simulink model "D2D_PHY_SI_Simulink"  (R2024b)
settings: Solver=VariableStepAuto  StartTime=0.0  StopTime=10.0  RelTol=1e-3
model workspace (MAT data in the model file):
  d2dCfg.link.modulation = 'PAM4'
  d2dCfg.link.baud_Gbps = 56.25
  d2dCfg.link.sps = 16
  d2dCfg.link.nBits = 10000
  d2dCfg.link.skipUI = 32
  d2dCfg.link.snr_dB = 28
  d2dCfg.link.rjUI_rms = 0.005
  d2dCfg.link.djUI_pp = 0.02
  d2dCfg.link.djFreq = 0.001
  d2dCfg.link.cdrBw = 0.1
  d2dCfg.link.seed = 202409
  d2dCfg.link.lineRate_Gbps = 112.5
  d2dCfg.link.baud_GBd = 56.25
  d2dCfg.rawPcs.pattern = 'PRBS31'
  d2dCfg.rawPcs.errInject = 0
  d2dCfg.txPma.lane.txEqMain = 0.98
  d2dCfg.txPma.lane.txEqPre = 0.01
  d2dCfg.txPma.lane.txEqPost = 0.01
  d2dCfg.txPma.lane.ffeNormalize = 1
  d2dCfg.txPma.lane.amplitude = 1
  d2dCfg.txPma.lane.ffeMode = 'three_tap'
  d2dCfg.txPma.lane.ffeOffsets = [-1 0 1]
  d2dCfg.txPma.lane.ffeCoeffs = [-0.01 0.98 -0.01]
  d2dCfg.txPma.lane.ffeCurrentConstraint = 1
  d2dCfg.txPma.lane.ffe.mode = 'three_tap'
  d2dCfg.txPma.lane.ffe.offsets = [-1 0 1]
  d2dCfg.txPma.lane.ffe.coeffs = [-0.01 0.98 -0.01]
  d2dCfg.txPma.lane.ffe.normalize = 1
  d2dCfg.txPma.lane.ffe.currentConstraint = 1
  d2dCfg.txPma.lane.sixTapPreset.offsets = [-2 -1 0 1 2 3]
  d2dCfg.txPma.lane.sixTapPreset.coeffs = [-0.03 -0.05 0.88 -0.06 -0.04 -0.02]
  d2dCfg.txPma.lane.sixTapPreset.description = 'model-selected regression assumption; not paper-disclosed coefficients'
  d2dCfg.txPma.lane.enableDacQuantization = 1
  d2dCfg.txPma.lane.dacLevels = 206
  d2dCfg.txPma.lane.targetSwing = 1
  d2dCfg.txPma.lane.gainError = 0
  d2dCfg.txPma.lane.enableSwingCalibration = 1
  d2dCfg.rxPma.lane.ctleBoost_dB = 4
  d2dCfg.rxPma.lane.ctleFz = 0.25
  d2dCfg.rxPma.lane.termGain = 1
  d2dCfg.rxPma.lane.clockMode = 'forwarded'
  d2dCfg.rxPma.lane.terminationMode = 'AC'
  d2dCfg.rxPma.lane.enableAcPre = 1
  d2dCfg.rxPma.lane.enableAcPost = 1
  d2dCfg.rxPma.lane.acPreCorner_UI = 0.0003
  d2dCfg.rxPma.lane.acPostCorner_UI = 0.0003
  d2dCfg.rxPma.lane.acInitialState = 'steady_state'
  d2dCfg.rxPma.lane.enableAgc = 0
  d2dCfg.rxPma.lane.ctlePolicy = 'paper_grid'
  d2dCfg.rxPma.lane.ctleGrid_dB = [0 0.2 0.4 0.6 0.8 1 1.2 1.4 1.6 1.8 2 2.2 2.4 2.6 2.8 3 3.2 3.4 3.6 3.8 4 4.2 4.4 4.6 4.8 5 5.2 5.4 5.6 5.8 6]
  d2dCfg.rxPma.lane.ctleAppliedBoost_dB = 4
  d2dCfg.rxPma.lane.samplerRoles.enabled = 1
  d2dCfg.rxPma.lane.samplerRoles.quarterRateBranches = 4
  d2dCfg.rxPma.lane.samplerRoles.roleCounts.data = 12
  d2dCfg.rxPma.lane.samplerRoles.roleCounts.edge = 4
  d2dCfg.rxPma.lane.samplerRoles.roleCounts.spare = 4
  d2dCfg.rxPma.lane.samplerRoles.roleCounts.total = 20
  d2dCfg.rxPma.lane.samplerRoles.levelShiftCodes.data = [2 0 -2]
  d2dCfg.rxPma.lane.samplerRoles.levelShiftCodes.edge = 0
  d2dCfg.rxPma.lane.samplerRoles.levelShiftCodes.spare = [3 1 -1 -3]
  d2dCfg.rxPma.lane.samplerRoles.samplerOffsetCodes = 0
  d2dCfg.rxPma.lane.samplerRoles.thresholdAssumptions = [-2 0 2]
  d2dCfg.rxPma.lane.samplerRoles.offsetCalibrationPlaceholder = 'not implemented in Stage D'
  d2dCfg.rxPma.lane.acSelectedCorner_UI = 0.0003
  d2dCfg.rxPma.lane.acSelectionBasis = 'bounded cycles/UI sweep; maximize valid received eye margin; no BER optimization'
  d2dCfg.channel.lossNyq_dB = 8
  d2dCfg.channel.poles = 3
  d2dCfg.channel.mode = 'analytic_il'
  d2dCfg.channel.refFreq_GHz = 28
  d2dCfg.channel.baud_GBd = 56.25
  d2dCfg.channel.lossAtRef_dB = 8
  d2dCfg.channel.lossSweep_dB = [0.5 2 4 6 8 10]
  d2dCfg.paper.id = 'VLSI2024_XSR_3nm'
  d2dCfg.paper.preset = 'VLSI Typical'
  d2dCfg.paper.mode = 'link_behavioral'
  d2dCfg.paper.rateRange_Gbps = [9.8 113]
  d2dCfg.paper.txEyeRate_Gbps = 112.5
  d2dCfg.paper.berRate_Gbps = 112
  d2dCfg.paper.headlineRate_Gbps = 113
  d2dCfg.paper.rateContext.range_Gbps = [9.8 113]
  d2dCfg.paper.rateContext.txEye_Gbps = 112.5
  d2dCfg.paper.rateContext.ber_Gbps = 112
  d2dCfg.paper.rateContext.headlineTable_Gbps = 113
  d2dCfg.paper.facts.packageTopology = '2D/2.5D CoWoS'
  d2dCfg.paper.facts.channelLength_mm = [1 80]
  d2dCfg.paper.facts.nextAt28GHz_dB = -40
  d2dCfg.paper.facts.fextAt28GHz_dB = -38
  d2dCfg.paper.facts.next_dB = -40
  d2dCfg.paper.facts.fext_dB = -38
  d2dCfg.paper.facts.quotedEnergy_pJ_per_bit = 0.9
  d2dCfg.paper.facts.dacLevels = 206
  d2dCfg.paper.facts.energy_pJ_per_bit = 0.9
  d2dCfg.paper.facts.ctleMaxBoost_dB = 6
  d2dCfg.paper.facts.ctleMaxStep_dB = 0.2
  d2dCfg.paper.facts.samplerRoleCounts.data = 12
  d2dCfg.paper.facts.samplerRoleCounts.edge = 4
  d2dCfg.paper.facts.samplerRoleCounts.spare = 4
  d2dCfg.paper.facts.samplerRoleCounts.total = 20
  d2dCfg.paper.facts.dllCount = 2
  d2dCfg.paper.facts.piCount = 1
  d2dCfg.paper.facts.piInlDnl = '< +/-0.5 LSB'
  d2dCfg.paper.facts.piInlDnl_LSB = '< +/-0.5 LSB'
  d2dCfg.paper.facts.pllTxIntegratedJitter_fs = 194
  d2dCfg.paper.facts.pllTxIntegratedJitter_UI = 0.0109125
  d2dCfg.paper.facts.pllTxIntegratedJitterContext = 'PLL+TX integrated; filter/measurement context'
  d2dCfg.paper.facts.table1LossAtRef_dB = 10.8
  d2dCfg.paper.facts.table1Loss_dB = 10.8
  d2dCfg.paper.facts.table1_IL_dB = 10.8
  d2dCfg.paper.assumptions.channelModel = 'calibrated analytic_il at 28 GHz; no real S-parameters'
  d2dCfg.paper.assumptions.quotedEnergyScope = 'quoted only; not a model prediction'
  d2dCfg.paper.assumptions.crosstalk = 'NEXT/FEXT facts recorded; MIMO crosstalk unmodeled'
  d2dCfg.phy.nLane = 8
  d2dCfg.model.useReferenceAlign = 0
  d2dCfg.model.useManualPhase = 0
  d2dCfg.model.manualPhaseUI = 0.5
  d2dCfg.model.manualDelayUI = 0
  d2dCfg.model.enablePaperAdaptation = 0
  d2dCfg.model.trainingMode = 'decision_directed'
  d2dCfg.model.cdrOptions.nCodes = 64
  d2dCfg.model.cdrOptions.initialPhaseUI = 0.5
  d2dCfg.model.cdrOptions.loopGainCodes = 1
  d2dCfg.model.cdrOptions.loopBandwidthProxy = 0.015625
  d2dCfg.model.cdrOptions.updateCadence = 1
  d2dCfg.model.cdrOptions.lockWindow = 32
  d2dCfg.model.cdrOptions.lockToleranceUI = 0.08
  d2dCfg.model.cdrOptions.mismatchBoundLSB = 0.49
  d2dCfg.model.cdrOptions.mismatchSeed = 202409
  d2dCfg.model.cdrOptions.enabled = 1
  d2dCfg.model.cdrOptions.maxStepCodes = 2
  d2dCfg.model.debugStages.startupCalibration = 1
  d2dCfg.model.debugStages.ctleTraining = 1
  d2dCfg.model.debugStages.ffeTraining = 1
  d2dCfg.model.debugStages.samplerCalibration = 1
  d2dCfg.model.debugStages.clockTraining = 1
  d2dCfg.model.debugStages.cdrEnabled = 1
  d2dCfg.model.debugStages.startupCalibrationBudgetUI = 64
  d2dCfg.model.debugStages.ctleTrainingBudgetUI = 128
  d2dCfg.model.debugStages.ffeTrainingBudgetUI = 128
  d2dCfg.model.debugStages.samplerCalibrationBudgetUI = 64
  d2dCfg.model.debugStages.clockTrainingBudgetUI = 64
  d2dCfg.model.debugStages.postLockWaitUI = 16
  d2dCfg.model.debugOptions.postLockWaitUI = 16
  d2dCfg.model.debugOptions.preLockSentinel = NaN
  d2dCfg.model.resultRoot = 'results/vlsi2024_xsr'
undefined symbols (not defined in the file or in its folder): dspChannel, dspCtle, dspFfeVector, dspMap, dspPam4Leveling, dspPaperCdr, dspPaperDriver, dspSample, dspSlice, repelem
settings Model: Creator=ahu161  LastModifiedBy=ahu161

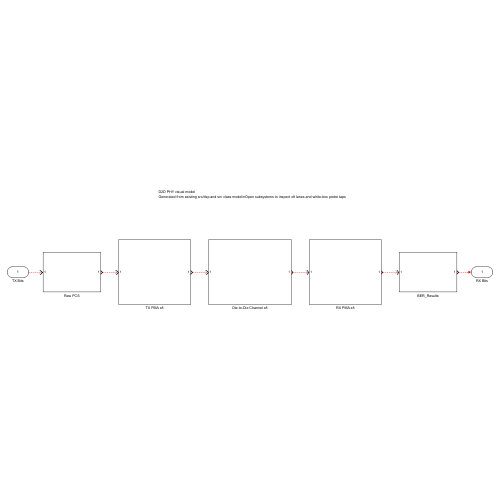
[thumbnail: Simulink's stored preview of the top-level diagram]
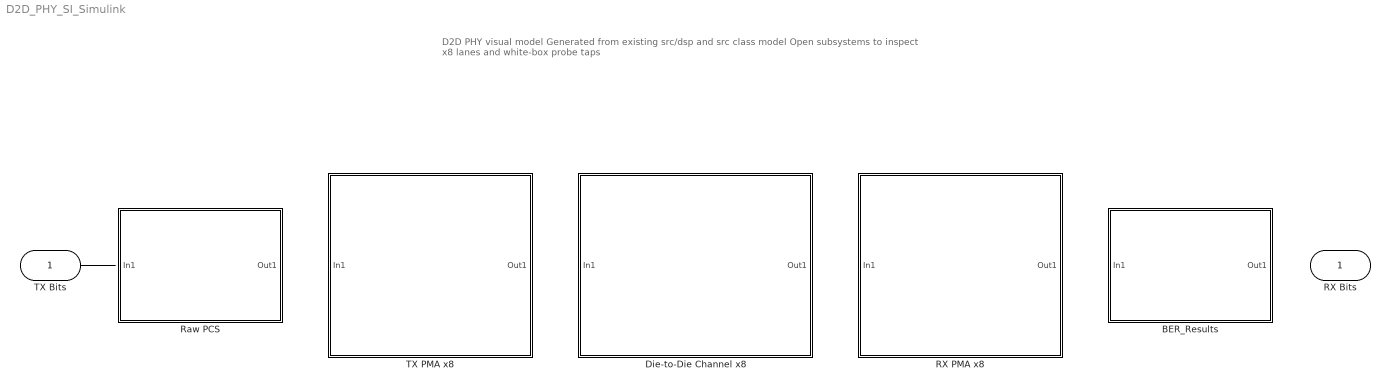
== system D2D_PHY_SI_Simulink ==
  note: D2D PHY visual model
      | Generated from existing src/dsp and src class model\nOpen subsystems to inspect x8 lanes and white-box probe taps
  TX Bits : Inport
  BER_Results : Subsystem
  Die-to-Die Channel x8 : Subsystem
  RX PMA x8 : Subsystem
  Raw PCS : Subsystem
  TX PMA x8 : Subsystem
  RX Bits : Outport
  wires:
  TX Bits/1 -> ?
  ? -> ?
  ? -> ?
  ? -> ?
  ? -> ?
  ? -> RX Bits/1

== system D2D_PHY_SI_Simulink/BER_Results ==
  In1 : Inport
  BER calculator : MATLABFcn  MATLABFcn=mean(u~=0)
  BER result : ToWorkspace  VariableName=simulinkBer  SampleTime=-1
  Out1 : Outport
  wires:
  In1/1 -> BER calculator/1
  BER calculator/1 -> BER result/1, Out1/1

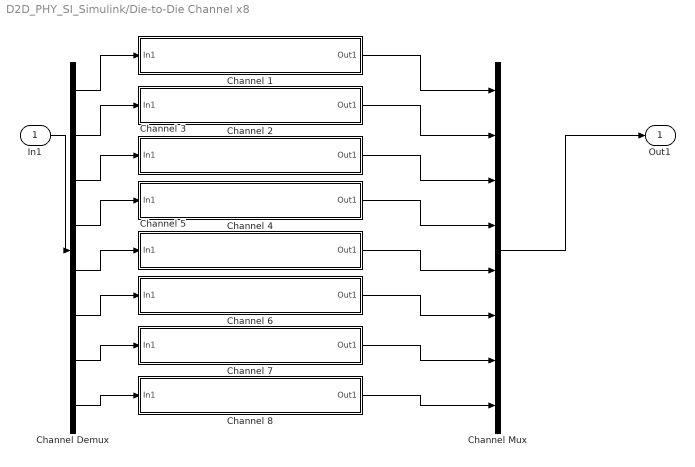
== system D2D_PHY_SI_Simulink/Die-to-Die Channel x8 ==
  In1 : Inport
  Channel 1 : Subsystem
  Channel 2 : Subsystem
  Channel 3 : Subsystem
  Channel 4 : Subsystem
  Channel 5 : Subsystem
  Channel 6 : Subsystem
  Channel 7 : Subsystem
  Channel 8 : Subsystem
  Channel Demux : Demux  Outputs=8
  Channel Mux : Mux  Inputs=8
  Out1 : Outport
  wires:
  In1/1 -> Channel Demux/1
  Channel Demux/1 -> Channel 1/1(In1)
  Channel 1/1(Out1) -> Channel Mux/1
  Channel Demux/2 -> Channel 2/1(In1)
  Channel 2/1(Out1) -> Channel Mux/2
  Channel Demux/3 -> Channel 3/1(In1)
  Channel 3/1(Out1) -> Channel Mux/3
  Channel Demux/4 -> Channel 4/1(In1)
  Channel 4/1(Out1) -> Channel Mux/4
  Channel Demux/5 -> Channel 5/1(In1)
  Channel 5/1(Out1) -> Channel Mux/5
  Channel Demux/6 -> Channel 6/1(In1)
  Channel 6/1(Out1) -> Channel Mux/6
  Channel Demux/7 -> Channel 7/1(In1)
  Channel 7/1(Out1) -> Channel Mux/7
  Channel Demux/8 -> Channel 8/1(In1)
  Channel 8/1(Out1) -> Channel Mux/8
  Channel Mux/1 -> Out1/1

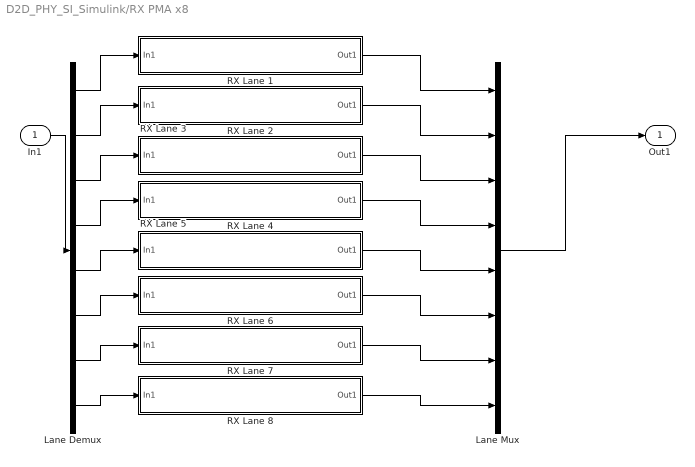
== system D2D_PHY_SI_Simulink/RX PMA x8 ==
  In1 : Inport
  Lane Demux : Demux  Outputs=8
  Lane Mux : Mux  Inputs=8
  RX Lane 1 : Subsystem
  RX Lane 2 : Subsystem
  RX Lane 3 : Subsystem
  RX Lane 4 : Subsystem
  RX Lane 5 : Subsystem
  RX Lane 6 : Subsystem
  RX Lane 7 : Subsystem
  RX Lane 8 : Subsystem
  Out1 : Outport
  wires:
  In1/1 -> Lane Demux/1
  Lane Demux/1 -> RX Lane 1/1(In1)
  RX Lane 1/1(Out1) -> Lane Mux/1
  Lane Demux/2 -> RX Lane 2/1(In1)
  RX Lane 2/1(Out1) -> Lane Mux/2
  Lane Demux/3 -> RX Lane 3/1(In1)
  RX Lane 3/1(Out1) -> Lane Mux/3
  Lane Demux/4 -> RX Lane 4/1(In1)
  RX Lane 4/1(Out1) -> Lane Mux/4
  Lane Demux/5 -> RX Lane 5/1(In1)
  RX Lane 5/1(Out1) -> Lane Mux/5
  Lane Demux/6 -> RX Lane 6/1(In1)
  RX Lane 6/1(Out1) -> Lane Mux/6
  Lane Demux/7 -> RX Lane 7/1(In1)
  RX Lane 7/1(Out1) -> Lane Mux/7
  Lane Demux/8 -> RX Lane 8/1(In1)
  RX Lane 8/1(Out1) -> Lane Mux/8
  Lane Mux/1 -> Out1/1

== system D2D_PHY_SI_Simulink/Raw PCS ==
  In1 : Inport
  dspPrbs_Pattern_Source : MATLABFcn  MATLABFcn=dspMap(u,d2dCfg.link.modulation)
  Out1 : Outport
  wires:
  In1/1 -> dspPrbs_Pattern_Source/1
  dspPrbs_Pattern_Source/1 -> [rawPcs_rxBits], Out1/1

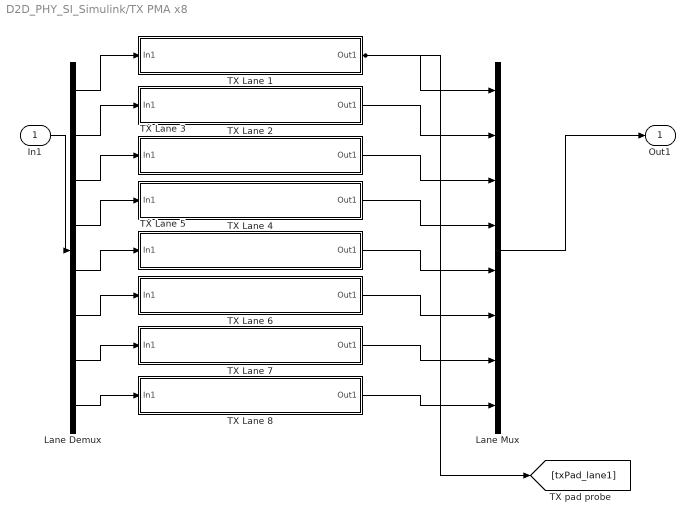
== system D2D_PHY_SI_Simulink/TX PMA x8 ==
  In1 : Inport
  Lane Demux : Demux  Outputs=8
  Lane Mux : Mux  Inputs=8
  TX Lane 1 : Subsystem
  TX Lane 2 : Subsystem
  TX Lane 3 : Subsystem
  TX Lane 4 : Subsystem
  TX Lane 5 : Subsystem
  TX Lane 6 : Subsystem
  TX Lane 7 : Subsystem
  TX Lane 8 : Subsystem
  Out1 : Outport
  wires:
  In1/1 -> Lane Demux/1
  Lane Demux/1 -> TX Lane 1/1(In1)
  TX Lane 1/1(Out1) -> Lane Mux/1, [txPad_lane1]
  Lane Demux/2 -> TX Lane 2/1(In1)
  TX Lane 2/1(Out1) -> Lane Mux/2
  Lane Demux/3 -> TX Lane 3/1(In1)
  TX Lane 3/1(Out1) -> Lane Mux/3
  Lane Demux/4 -> TX Lane 4/1(In1)
  TX Lane 4/1(Out1) -> Lane Mux/4
  Lane Demux/5 -> TX Lane 5/1(In1)
  TX Lane 5/1(Out1) -> Lane Mux/5
  Lane Demux/6 -> TX Lane 6/1(In1)
  TX Lane 6/1(Out1) -> Lane Mux/6
  Lane Demux/7 -> TX Lane 7/1(In1)
  TX Lane 7/1(Out1) -> Lane Mux/7
  Lane Demux/8 -> TX Lane 8/1(In1)
  TX Lane 8/1(Out1) -> Lane Mux/8
  Lane Mux/1 -> Out1/1

== system D2D_PHY_SI_Simulink/Die-to-Die Channel x8/Channel 1 ==
  In1 : Inport
  dspChannel : MATLABFcn  MATLABFcn=dspChannel(u,d2dCfg.link.sps,d2dCfg.channel.lossAtRef_dB,d2dCfg.channel.poles,struct('mode',d2dCfg.channel.mode,'refFreq_GHz',d2dCfg.channel.refFreq_GHz,'baud_GBd',d2dCfg.channel.baud_GBd,'lossAtRef_dB',d2dCfg.channel.lossAtRef_dB))
  Out1 : Outport
  wires:
  In1/1 -> dspChannel/1
  dspChannel/1 -> Out1/1

== system D2D_PHY_SI_Simulink/Die-to-Die Channel x8/Channel 2 ==
  In1 : Inport
  dspChannel : MATLABFcn  MATLABFcn=dspChannel(u,d2dCfg.link.sps,d2dCfg.channel.lossAtRef_dB,d2dCfg.channel.poles,struct('mode',d2dCfg.channel.mode,'refFreq_GHz',d2dCfg.channel.refFreq_GHz,'baud_GBd',d2dCfg.channel.baud_GBd,'lossAtRef_dB',d2dCfg.channel.lossAtRef_dB))
  Out1 : Outport
  wires:
  In1/1 -> dspChannel/1
  dspChannel/1 -> Out1/1

== system D2D_PHY_SI_Simulink/Die-to-Die Channel x8/Channel 3 ==
  In1 : Inport
  dspChannel : MATLABFcn  MATLABFcn=dspChannel(u,d2dCfg.link.sps,d2dCfg.channel.lossAtRef_dB,d2dCfg.channel.poles,struct('mode',d2dCfg.channel.mode,'refFreq_GHz',d2dCfg.channel.refFreq_GHz,'baud_GBd',d2dCfg.channel.baud_GBd,'lossAtRef_dB',d2dCfg.channel.lossAtRef_dB))
  Out1 : Outport
  wires:
  In1/1 -> dspChannel/1
  dspChannel/1 -> Out1/1

== system D2D_PHY_SI_Simulink/Die-to-Die Channel x8/Channel 4 ==
  In1 : Inport
  dspChannel : MATLABFcn  MATLABFcn=dspChannel(u,d2dCfg.link.sps,d2dCfg.channel.lossAtRef_dB,d2dCfg.channel.poles,struct('mode',d2dCfg.channel.mode,'refFreq_GHz',d2dCfg.channel.refFreq_GHz,'baud_GBd',d2dCfg.channel.baud_GBd,'lossAtRef_dB',d2dCfg.channel.lossAtRef_dB))
  Out1 : Outport
  wires:
  In1/1 -> dspChannel/1
  dspChannel/1 -> Out1/1

== system D2D_PHY_SI_Simulink/Die-to-Die Channel x8/Channel 5 ==
  In1 : Inport
  dspChannel : MATLABFcn  MATLABFcn=dspChannel(u,d2dCfg.link.sps,d2dCfg.channel.lossAtRef_dB,d2dCfg.channel.poles,struct('mode',d2dCfg.channel.mode,'refFreq_GHz',d2dCfg.channel.refFreq_GHz,'baud_GBd',d2dCfg.channel.baud_GBd,'lossAtRef_dB',d2dCfg.channel.lossAtRef_dB))
  Out1 : Outport
  wires:
  In1/1 -> dspChannel/1
  dspChannel/1 -> Out1/1

== system D2D_PHY_SI_Simulink/Die-to-Die Channel x8/Channel 6 ==
  In1 : Inport
  dspChannel : MATLABFcn  MATLABFcn=dspChannel(u,d2dCfg.link.sps,d2dCfg.channel.lossAtRef_dB,d2dCfg.channel.poles,struct('mode',d2dCfg.channel.mode,'refFreq_GHz',d2dCfg.channel.refFreq_GHz,'baud_GBd',d2dCfg.channel.baud_GBd,'lossAtRef_dB',d2dCfg.channel.lossAtRef_dB))
  Out1 : Outport
  wires:
  In1/1 -> dspChannel/1
  dspChannel/1 -> Out1/1

== system D2D_PHY_SI_Simulink/Die-to-Die Channel x8/Channel 7 ==
  In1 : Inport
  dspChannel : MATLABFcn  MATLABFcn=dspChannel(u,d2dCfg.link.sps,d2dCfg.channel.lossAtRef_dB,d2dCfg.channel.poles,struct('mode',d2dCfg.channel.mode,'refFreq_GHz',d2dCfg.channel.refFreq_GHz,'baud_GBd',d2dCfg.channel.baud_GBd,'lossAtRef_dB',d2dCfg.channel.lossAtRef_dB))
  Out1 : Outport
  wires:
  In1/1 -> dspChannel/1
  dspChannel/1 -> Out1/1

== system D2D_PHY_SI_Simulink/Die-to-Die Channel x8/Channel 8 ==
  In1 : Inport
  dspChannel : MATLABFcn  MATLABFcn=dspChannel(u,d2dCfg.link.sps,d2dCfg.channel.lossAtRef_dB,d2dCfg.channel.poles,struct('mode',d2dCfg.channel.mode,'refFreq_GHz',d2dCfg.channel.refFreq_GHz,'baud_GBd',d2dCfg.channel.baud_GBd,'lossAtRef_dB',d2dCfg.channel.lossAtRef_dB))
  Out1 : Outport
  wires:
  In1/1 -> dspChannel/1
  dspChannel/1 -> Out1/1

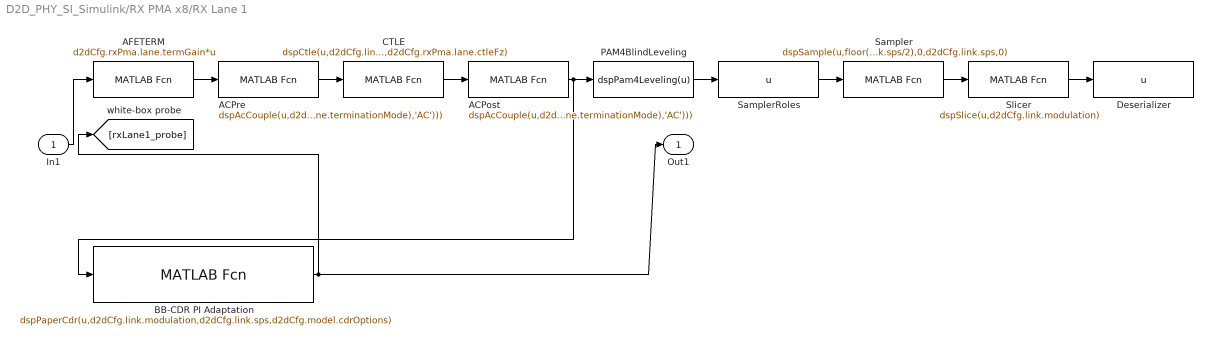
== system D2D_PHY_SI_Simulink/RX PMA x8/RX Lane 1 ==
  In1 : Inport
  ACPost : MATLABFcn  MATLABFcn=dspAcCouple(u,d2dCfg.link.sps,d2dCfg.rxPma.lane.acPostCorner_UI,struct('enabled',d2dCfg.rxPma.lane.enableAcPost && strcmpi(char(d2dCfg.rxPma.lane.terminationMode),'AC')))
  ACPre : MATLABFcn  MATLABFcn=dspAcCouple(u,d2dCfg.link.sps,d2dCfg.rxPma.lane.acPreCorner_UI,struct('enabled',d2dCfg.rxPma.lane.enableAcPre && strcmpi(char(d2dCfg.rxPma.lane.terminationMode),'AC')))
  AFETERM : MATLABFcn  MATLABFcn=d2dCfg.rxPma.lane.termGain*u
  BB-CDR PI Adaptation : MATLABFcn  MATLABFcn=dspPaperCdr(u,d2dCfg.link.modulation,d2dCfg.link.sps,d2dCfg.model.cdrOptions)
  CTLE : MATLABFcn  MATLABFcn=dspCtle(u,d2dCfg.link.sps,d2dCfg.rxPma.lane.ctleBoost_dB,d2dCfg.rxPma.lane.ctleFz)
  Deserializer : MATLABFcn  MATLABFcn=u
  PAM4BlindLeveling : MATLABFcn  MATLABFcn=dspPam4Leveling(u)
  Sampler : MATLABFcn  MATLABFcn=dspSample(u,floor(d2dCfg.link.sps/2),0,d2dCfg.link.sps,0)
  SamplerRoles : MATLABFcn  MATLABFcn=u
  Slicer : MATLABFcn  MATLABFcn=dspSlice(u,d2dCfg.link.modulation)
  Out1 : Outport
  wires:
  In1/1 -> AFETERM/1
  AFETERM/1 -> ACPre/1
  ACPre/1 -> CTLE/1
  CTLE/1 -> ACPost/1
  ACPost/1 -> PAM4BlindLeveling/1, BB-CDR PI Adaptation/1
  PAM4BlindLeveling/1 -> SamplerRoles/1
  SamplerRoles/1 -> Sampler/1
  Sampler/1 -> Slicer/1
  Slicer/1 -> Deserializer/1
  BB-CDR PI Adaptation/1 -> Out1/1, [rxLane1_probe]

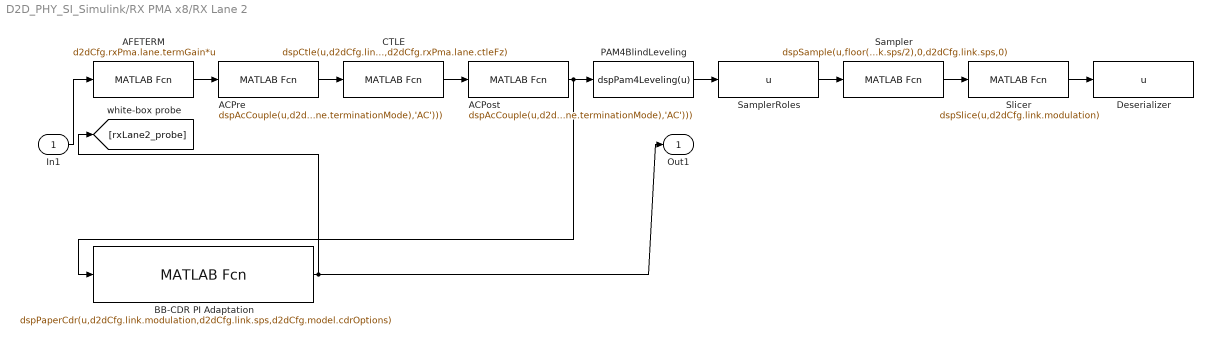
== system D2D_PHY_SI_Simulink/RX PMA x8/RX Lane 2 ==
  In1 : Inport
  ACPost : MATLABFcn  MATLABFcn=dspAcCouple(u,d2dCfg.link.sps,d2dCfg.rxPma.lane.acPostCorner_UI,struct('enabled',d2dCfg.rxPma.lane.enableAcPost && strcmpi(char(d2dCfg.rxPma.lane.terminationMode),'AC')))
  ACPre : MATLABFcn  MATLABFcn=dspAcCouple(u,d2dCfg.link.sps,d2dCfg.rxPma.lane.acPreCorner_UI,struct('enabled',d2dCfg.rxPma.lane.enableAcPre && strcmpi(char(d2dCfg.rxPma.lane.terminationMode),'AC')))
  AFETERM : MATLABFcn  MATLABFcn=d2dCfg.rxPma.lane.termGain*u
  BB-CDR PI Adaptation : MATLABFcn  MATLABFcn=dspPaperCdr(u,d2dCfg.link.modulation,d2dCfg.link.sps,d2dCfg.model.cdrOptions)
  CTLE : MATLABFcn  MATLABFcn=dspCtle(u,d2dCfg.link.sps,d2dCfg.rxPma.lane.ctleBoost_dB,d2dCfg.rxPma.lane.ctleFz)
  Deserializer : MATLABFcn  MATLABFcn=u
  PAM4BlindLeveling : MATLABFcn  MATLABFcn=dspPam4Leveling(u)
  Sampler : MATLABFcn  MATLABFcn=dspSample(u,floor(d2dCfg.link.sps/2),0,d2dCfg.link.sps,0)
  SamplerRoles : MATLABFcn  MATLABFcn=u
  Slicer : MATLABFcn  MATLABFcn=dspSlice(u,d2dCfg.link.modulation)
  Out1 : Outport
  wires:
  In1/1 -> AFETERM/1
  AFETERM/1 -> ACPre/1
  ACPre/1 -> CTLE/1
  CTLE/1 -> ACPost/1
  ACPost/1 -> PAM4BlindLeveling/1, BB-CDR PI Adaptation/1
  PAM4BlindLeveling/1 -> SamplerRoles/1
  SamplerRoles/1 -> Sampler/1
  Sampler/1 -> Slicer/1
  Slicer/1 -> Deserializer/1
  BB-CDR PI Adaptation/1 -> Out1/1, [rxLane2_probe]

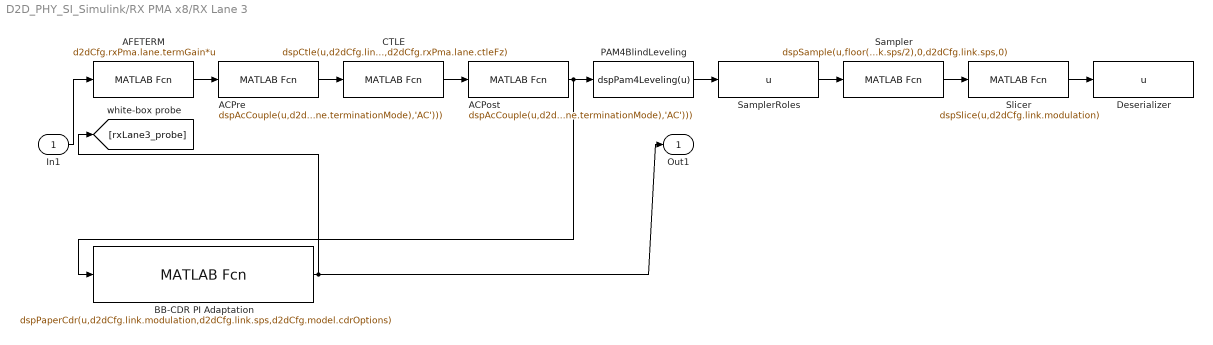
== system D2D_PHY_SI_Simulink/RX PMA x8/RX Lane 3 ==
  In1 : Inport
  ACPost : MATLABFcn  MATLABFcn=dspAcCouple(u,d2dCfg.link.sps,d2dCfg.rxPma.lane.acPostCorner_UI,struct('enabled',d2dCfg.rxPma.lane.enableAcPost && strcmpi(char(d2dCfg.rxPma.lane.terminationMode),'AC')))
  ACPre : MATLABFcn  MATLABFcn=dspAcCouple(u,d2dCfg.link.sps,d2dCfg.rxPma.lane.acPreCorner_UI,struct('enabled',d2dCfg.rxPma.lane.enableAcPre && strcmpi(char(d2dCfg.rxPma.lane.terminationMode),'AC')))
  AFETERM : MATLABFcn  MATLABFcn=d2dCfg.rxPma.lane.termGain*u
  BB-CDR PI Adaptation : MATLABFcn  MATLABFcn=dspPaperCdr(u,d2dCfg.link.modulation,d2dCfg.link.sps,d2dCfg.model.cdrOptions)
  CTLE : MATLABFcn  MATLABFcn=dspCtle(u,d2dCfg.link.sps,d2dCfg.rxPma.lane.ctleBoost_dB,d2dCfg.rxPma.lane.ctleFz)
  Deserializer : MATLABFcn  MATLABFcn=u
  PAM4BlindLeveling : MATLABFcn  MATLABFcn=dspPam4Leveling(u)
  Sampler : MATLABFcn  MATLABFcn=dspSample(u,floor(d2dCfg.link.sps/2),0,d2dCfg.link.sps,0)
  SamplerRoles : MATLABFcn  MATLABFcn=u
  Slicer : MATLABFcn  MATLABFcn=dspSlice(u,d2dCfg.link.modulation)
  Out1 : Outport
  wires:
  In1/1 -> AFETERM/1
  AFETERM/1 -> ACPre/1
  ACPre/1 -> CTLE/1
  CTLE/1 -> ACPost/1
  ACPost/1 -> PAM4BlindLeveling/1, BB-CDR PI Adaptation/1
  PAM4BlindLeveling/1 -> SamplerRoles/1
  SamplerRoles/1 -> Sampler/1
  Sampler/1 -> Slicer/1
  Slicer/1 -> Deserializer/1
  BB-CDR PI Adaptation/1 -> Out1/1, [rxLane3_probe]

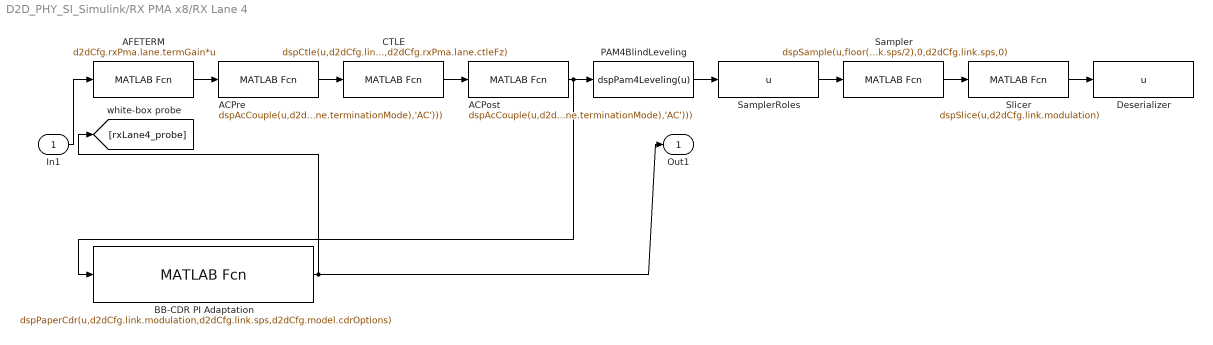
== system D2D_PHY_SI_Simulink/RX PMA x8/RX Lane 4 ==
  In1 : Inport
  ACPost : MATLABFcn  MATLABFcn=dspAcCouple(u,d2dCfg.link.sps,d2dCfg.rxPma.lane.acPostCorner_UI,struct('enabled',d2dCfg.rxPma.lane.enableAcPost && strcmpi(char(d2dCfg.rxPma.lane.terminationMode),'AC')))
  ACPre : MATLABFcn  MATLABFcn=dspAcCouple(u,d2dCfg.link.sps,d2dCfg.rxPma.lane.acPreCorner_UI,struct('enabled',d2dCfg.rxPma.lane.enableAcPre && strcmpi(char(d2dCfg.rxPma.lane.terminationMode),'AC')))
  AFETERM : MATLABFcn  MATLABFcn=d2dCfg.rxPma.lane.termGain*u
  BB-CDR PI Adaptation : MATLABFcn  MATLABFcn=dspPaperCdr(u,d2dCfg.link.modulation,d2dCfg.link.sps,d2dCfg.model.cdrOptions)
  CTLE : MATLABFcn  MATLABFcn=dspCtle(u,d2dCfg.link.sps,d2dCfg.rxPma.lane.ctleBoost_dB,d2dCfg.rxPma.lane.ctleFz)
  Deserializer : MATLABFcn  MATLABFcn=u
  PAM4BlindLeveling : MATLABFcn  MATLABFcn=dspPam4Leveling(u)
  Sampler : MATLABFcn  MATLABFcn=dspSample(u,floor(d2dCfg.link.sps/2),0,d2dCfg.link.sps,0)
  SamplerRoles : MATLABFcn  MATLABFcn=u
  Slicer : MATLABFcn  MATLABFcn=dspSlice(u,d2dCfg.link.modulation)
  Out1 : Outport
  wires:
  In1/1 -> AFETERM/1
  AFETERM/1 -> ACPre/1
  ACPre/1 -> CTLE/1
  CTLE/1 -> ACPost/1
  ACPost/1 -> PAM4BlindLeveling/1, BB-CDR PI Adaptation/1
  PAM4BlindLeveling/1 -> SamplerRoles/1
  SamplerRoles/1 -> Sampler/1
  Sampler/1 -> Slicer/1
  Slicer/1 -> Deserializer/1
  BB-CDR PI Adaptation/1 -> Out1/1, [rxLane4_probe]

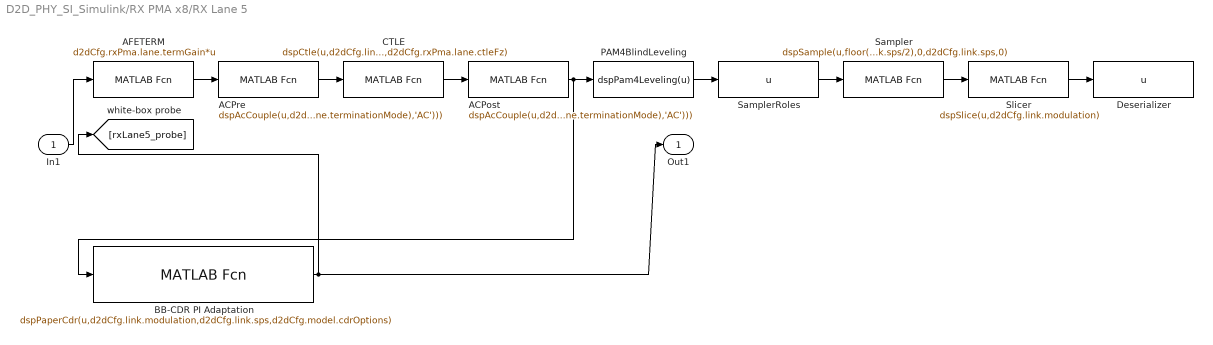
== system D2D_PHY_SI_Simulink/RX PMA x8/RX Lane 5 ==
  In1 : Inport
  ACPost : MATLABFcn  MATLABFcn=dspAcCouple(u,d2dCfg.link.sps,d2dCfg.rxPma.lane.acPostCorner_UI,struct('enabled',d2dCfg.rxPma.lane.enableAcPost && strcmpi(char(d2dCfg.rxPma.lane.terminationMode),'AC')))
  ACPre : MATLABFcn  MATLABFcn=dspAcCouple(u,d2dCfg.link.sps,d2dCfg.rxPma.lane.acPreCorner_UI,struct('enabled',d2dCfg.rxPma.lane.enableAcPre && strcmpi(char(d2dCfg.rxPma.lane.terminationMode),'AC')))
  AFETERM : MATLABFcn  MATLABFcn=d2dCfg.rxPma.lane.termGain*u
  BB-CDR PI Adaptation : MATLABFcn  MATLABFcn=dspPaperCdr(u,d2dCfg.link.modulation,d2dCfg.link.sps,d2dCfg.model.cdrOptions)
  CTLE : MATLABFcn  MATLABFcn=dspCtle(u,d2dCfg.link.sps,d2dCfg.rxPma.lane.ctleBoost_dB,d2dCfg.rxPma.lane.ctleFz)
  Deserializer : MATLABFcn  MATLABFcn=u
  PAM4BlindLeveling : MATLABFcn  MATLABFcn=dspPam4Leveling(u)
  Sampler : MATLABFcn  MATLABFcn=dspSample(u,floor(d2dCfg.link.sps/2),0,d2dCfg.link.sps,0)
  SamplerRoles : MATLABFcn  MATLABFcn=u
  Slicer : MATLABFcn  MATLABFcn=dspSlice(u,d2dCfg.link.modulation)
  Out1 : Outport
  wires:
  In1/1 -> AFETERM/1
  AFETERM/1 -> ACPre/1
  ACPre/1 -> CTLE/1
  CTLE/1 -> ACPost/1
  ACPost/1 -> PAM4BlindLeveling/1, BB-CDR PI Adaptation/1
  PAM4BlindLeveling/1 -> SamplerRoles/1
  SamplerRoles/1 -> Sampler/1
  Sampler/1 -> Slicer/1
  Slicer/1 -> Deserializer/1
  BB-CDR PI Adaptation/1 -> Out1/1, [rxLane5_probe]

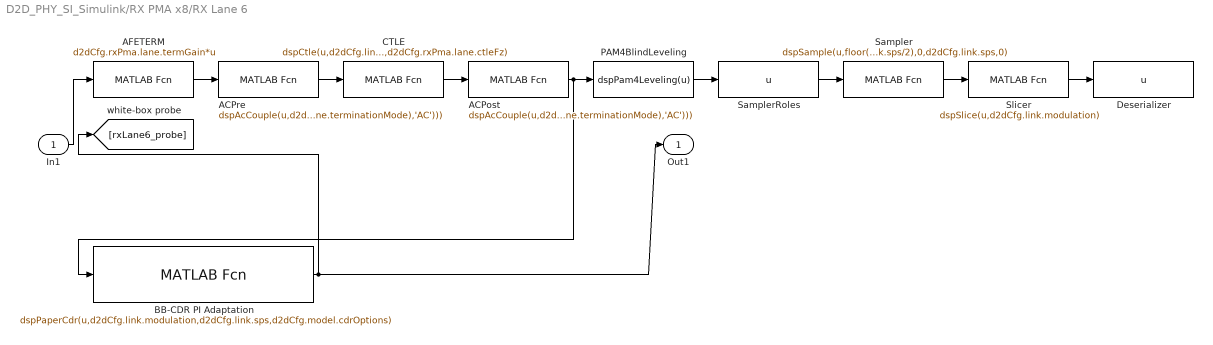
== system D2D_PHY_SI_Simulink/RX PMA x8/RX Lane 6 ==
  In1 : Inport
  ACPost : MATLABFcn  MATLABFcn=dspAcCouple(u,d2dCfg.link.sps,d2dCfg.rxPma.lane.acPostCorner_UI,struct('enabled',d2dCfg.rxPma.lane.enableAcPost && strcmpi(char(d2dCfg.rxPma.lane.terminationMode),'AC')))
  ACPre : MATLABFcn  MATLABFcn=dspAcCouple(u,d2dCfg.link.sps,d2dCfg.rxPma.lane.acPreCorner_UI,struct('enabled',d2dCfg.rxPma.lane.enableAcPre && strcmpi(char(d2dCfg.rxPma.lane.terminationMode),'AC')))
  AFETERM : MATLABFcn  MATLABFcn=d2dCfg.rxPma.lane.termGain*u
  BB-CDR PI Adaptation : MATLABFcn  MATLABFcn=dspPaperCdr(u,d2dCfg.link.modulation,d2dCfg.link.sps,d2dCfg.model.cdrOptions)
  CTLE : MATLABFcn  MATLABFcn=dspCtle(u,d2dCfg.link.sps,d2dCfg.rxPma.lane.ctleBoost_dB,d2dCfg.rxPma.lane.ctleFz)
  Deserializer : MATLABFcn  MATLABFcn=u
  PAM4BlindLeveling : MATLABFcn  MATLABFcn=dspPam4Leveling(u)
  Sampler : MATLABFcn  MATLABFcn=dspSample(u,floor(d2dCfg.link.sps/2),0,d2dCfg.link.sps,0)
  SamplerRoles : MATLABFcn  MATLABFcn=u
  Slicer : MATLABFcn  MATLABFcn=dspSlice(u,d2dCfg.link.modulation)
  Out1 : Outport
  wires:
  In1/1 -> AFETERM/1
  AFETERM/1 -> ACPre/1
  ACPre/1 -> CTLE/1
  CTLE/1 -> ACPost/1
  ACPost/1 -> PAM4BlindLeveling/1, BB-CDR PI Adaptation/1
  PAM4BlindLeveling/1 -> SamplerRoles/1
  SamplerRoles/1 -> Sampler/1
  Sampler/1 -> Slicer/1
  Slicer/1 -> Deserializer/1
  BB-CDR PI Adaptation/1 -> Out1/1, [rxLane6_probe]

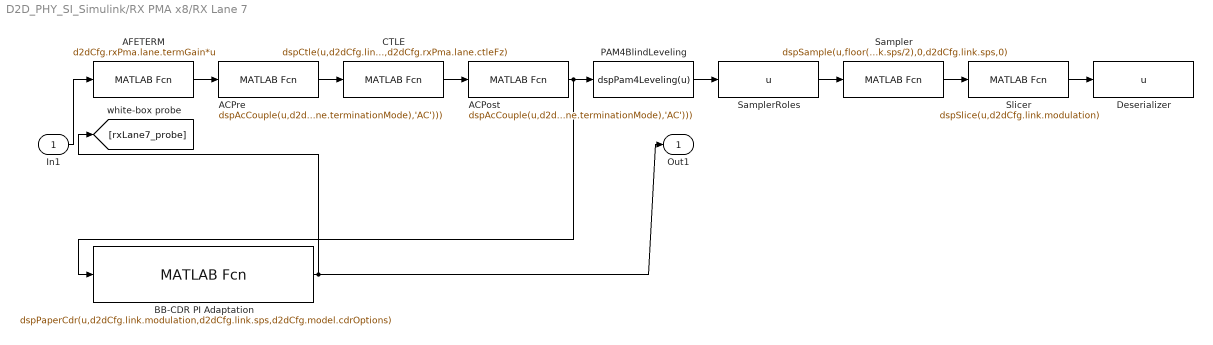
== system D2D_PHY_SI_Simulink/RX PMA x8/RX Lane 7 ==
  In1 : Inport
  ACPost : MATLABFcn  MATLABFcn=dspAcCouple(u,d2dCfg.link.sps,d2dCfg.rxPma.lane.acPostCorner_UI,struct('enabled',d2dCfg.rxPma.lane.enableAcPost && strcmpi(char(d2dCfg.rxPma.lane.terminationMode),'AC')))
  ACPre : MATLABFcn  MATLABFcn=dspAcCouple(u,d2dCfg.link.sps,d2dCfg.rxPma.lane.acPreCorner_UI,struct('enabled',d2dCfg.rxPma.lane.enableAcPre && strcmpi(char(d2dCfg.rxPma.lane.terminationMode),'AC')))
  AFETERM : MATLABFcn  MATLABFcn=d2dCfg.rxPma.lane.termGain*u
  BB-CDR PI Adaptation : MATLABFcn  MATLABFcn=dspPaperCdr(u,d2dCfg.link.modulation,d2dCfg.link.sps,d2dCfg.model.cdrOptions)
  CTLE : MATLABFcn  MATLABFcn=dspCtle(u,d2dCfg.link.sps,d2dCfg.rxPma.lane.ctleBoost_dB,d2dCfg.rxPma.lane.ctleFz)
  Deserializer : MATLABFcn  MATLABFcn=u
  PAM4BlindLeveling : MATLABFcn  MATLABFcn=dspPam4Leveling(u)
  Sampler : MATLABFcn  MATLABFcn=dspSample(u,floor(d2dCfg.link.sps/2),0,d2dCfg.link.sps,0)
  SamplerRoles : MATLABFcn  MATLABFcn=u
  Slicer : MATLABFcn  MATLABFcn=dspSlice(u,d2dCfg.link.modulation)
  Out1 : Outport
  wires:
  In1/1 -> AFETERM/1
  AFETERM/1 -> ACPre/1
  ACPre/1 -> CTLE/1
  CTLE/1 -> ACPost/1
  ACPost/1 -> PAM4BlindLeveling/1, BB-CDR PI Adaptation/1
  PAM4BlindLeveling/1 -> SamplerRoles/1
  SamplerRoles/1 -> Sampler/1
  Sampler/1 -> Slicer/1
  Slicer/1 -> Deserializer/1
  BB-CDR PI Adaptation/1 -> Out1/1, [rxLane7_probe]

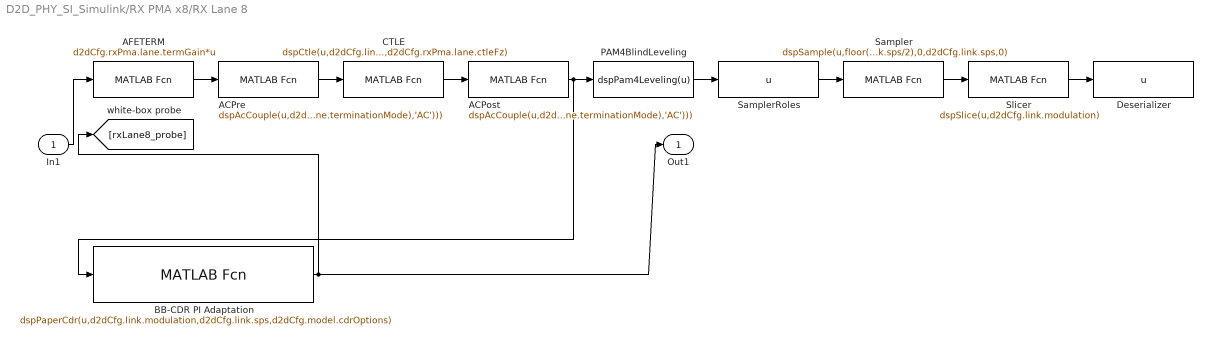
== system D2D_PHY_SI_Simulink/RX PMA x8/RX Lane 8 ==
  In1 : Inport
  ACPost : MATLABFcn  MATLABFcn=dspAcCouple(u,d2dCfg.link.sps,d2dCfg.rxPma.lane.acPostCorner_UI,struct('enabled',d2dCfg.rxPma.lane.enableAcPost && strcmpi(char(d2dCfg.rxPma.lane.terminationMode),'AC')))
  ACPre : MATLABFcn  MATLABFcn=dspAcCouple(u,d2dCfg.link.sps,d2dCfg.rxPma.lane.acPreCorner_UI,struct('enabled',d2dCfg.rxPma.lane.enableAcPre && strcmpi(char(d2dCfg.rxPma.lane.terminationMode),'AC')))
  AFETERM : MATLABFcn  MATLABFcn=d2dCfg.rxPma.lane.termGain*u
  BB-CDR PI Adaptation : MATLABFcn  MATLABFcn=dspPaperCdr(u,d2dCfg.link.modulation,d2dCfg.link.sps,d2dCfg.model.cdrOptions)
  CTLE : MATLABFcn  MATLABFcn=dspCtle(u,d2dCfg.link.sps,d2dCfg.rxPma.lane.ctleBoost_dB,d2dCfg.rxPma.lane.ctleFz)
  Deserializer : MATLABFcn  MATLABFcn=u
  PAM4BlindLeveling : MATLABFcn  MATLABFcn=dspPam4Leveling(u)
  Sampler : MATLABFcn  MATLABFcn=dspSample(u,floor(d2dCfg.link.sps/2),0,d2dCfg.link.sps,0)
  SamplerRoles : MATLABFcn  MATLABFcn=u
  Slicer : MATLABFcn  MATLABFcn=dspSlice(u,d2dCfg.link.modulation)
  Out1 : Outport
  wires:
  In1/1 -> AFETERM/1
  AFETERM/1 -> ACPre/1
  ACPre/1 -> CTLE/1
  CTLE/1 -> ACPost/1
  ACPost/1 -> PAM4BlindLeveling/1, BB-CDR PI Adaptation/1
  PAM4BlindLeveling/1 -> SamplerRoles/1
  SamplerRoles/1 -> Sampler/1
  Sampler/1 -> Slicer/1
  Slicer/1 -> Deserializer/1
  BB-CDR PI Adaptation/1 -> Out1/1, [rxLane8_probe]

== system D2D_PHY_SI_Simulink/TX PMA x8/TX Lane 1 ==
  In1 : Inport
  DAC_Driver : MATLABFcn  MATLABFcn=dspPaperDriver(u,d2dCfg.txPma.lane)
  FFEVector : MATLABFcn  MATLABFcn=dspFfeVector(u,d2dCfg.txPma.lane.ffeCoeffs,d2dCfg.txPma.lane.ffeOffsets,struct('normalize',d2dCfg.txPma.lane.ffeNormalize,'currentConstraint',d2dCfg.txPma.lane.ffeCurrentConstraint))
  Serializer : MATLABFcn  MATLABFcn=repelem(u,d2dCfg.link.sps)
  Out1 : Outport
  wires:
  In1/1 -> FFEVector/1
  FFEVector/1 -> Serializer/1
  Serializer/1 -> DAC_Driver/1
  DAC_Driver/1 -> Out1/1, [txLane1_probe]

== system D2D_PHY_SI_Simulink/TX PMA x8/TX Lane 2 ==
  In1 : Inport
  DAC_Driver : MATLABFcn  MATLABFcn=dspPaperDriver(u,d2dCfg.txPma.lane)
  FFEVector : MATLABFcn  MATLABFcn=dspFfeVector(u,d2dCfg.txPma.lane.ffeCoeffs,d2dCfg.txPma.lane.ffeOffsets,struct('normalize',d2dCfg.txPma.lane.ffeNormalize,'currentConstraint',d2dCfg.txPma.lane.ffeCurrentConstraint))
  Serializer : MATLABFcn  MATLABFcn=repelem(u,d2dCfg.link.sps)
  Out1 : Outport
  wires:
  In1/1 -> FFEVector/1
  FFEVector/1 -> Serializer/1
  Serializer/1 -> DAC_Driver/1
  DAC_Driver/1 -> Out1/1, [txLane2_probe]

== system D2D_PHY_SI_Simulink/TX PMA x8/TX Lane 3 ==
  In1 : Inport
  DAC_Driver : MATLABFcn  MATLABFcn=dspPaperDriver(u,d2dCfg.txPma.lane)
  FFEVector : MATLABFcn  MATLABFcn=dspFfeVector(u,d2dCfg.txPma.lane.ffeCoeffs,d2dCfg.txPma.lane.ffeOffsets,struct('normalize',d2dCfg.txPma.lane.ffeNormalize,'currentConstraint',d2dCfg.txPma.lane.ffeCurrentConstraint))
  Serializer : MATLABFcn  MATLABFcn=repelem(u,d2dCfg.link.sps)
  Out1 : Outport
  wires:
  In1/1 -> FFEVector/1
  FFEVector/1 -> Serializer/1
  Serializer/1 -> DAC_Driver/1
  DAC_Driver/1 -> Out1/1, [txLane3_probe]

== system D2D_PHY_SI_Simulink/TX PMA x8/TX Lane 4 ==
  In1 : Inport
  DAC_Driver : MATLABFcn  MATLABFcn=dspPaperDriver(u,d2dCfg.txPma.lane)
  FFEVector : MATLABFcn  MATLABFcn=dspFfeVector(u,d2dCfg.txPma.lane.ffeCoeffs,d2dCfg.txPma.lane.ffeOffsets,struct('normalize',d2dCfg.txPma.lane.ffeNormalize,'currentConstraint',d2dCfg.txPma.lane.ffeCurrentConstraint))
  Serializer : MATLABFcn  MATLABFcn=repelem(u,d2dCfg.link.sps)
  Out1 : Outport
  wires:
  In1/1 -> FFEVector/1
  FFEVector/1 -> Serializer/1
  Serializer/1 -> DAC_Driver/1
  DAC_Driver/1 -> Out1/1, [txLane4_probe]

== system D2D_PHY_SI_Simulink/TX PMA x8/TX Lane 5 ==
  In1 : Inport
  DAC_Driver : MATLABFcn  MATLABFcn=dspPaperDriver(u,d2dCfg.txPma.lane)
  FFEVector : MATLABFcn  MATLABFcn=dspFfeVector(u,d2dCfg.txPma.lane.ffeCoeffs,d2dCfg.txPma.lane.ffeOffsets,struct('normalize',d2dCfg.txPma.lane.ffeNormalize,'currentConstraint',d2dCfg.txPma.lane.ffeCurrentConstraint))
  Serializer : MATLABFcn  MATLABFcn=repelem(u,d2dCfg.link.sps)
  Out1 : Outport
  wires:
  In1/1 -> FFEVector/1
  FFEVector/1 -> Serializer/1
  Serializer/1 -> DAC_Driver/1
  DAC_Driver/1 -> Out1/1, [txLane5_probe]

== system D2D_PHY_SI_Simulink/TX PMA x8/TX Lane 6 ==
  In1 : Inport
  DAC_Driver : MATLABFcn  MATLABFcn=dspPaperDriver(u,d2dCfg.txPma.lane)
  FFEVector : MATLABFcn  MATLABFcn=dspFfeVector(u,d2dCfg.txPma.lane.ffeCoeffs,d2dCfg.txPma.lane.ffeOffsets,struct('normalize',d2dCfg.txPma.lane.ffeNormalize,'currentConstraint',d2dCfg.txPma.lane.ffeCurrentConstraint))
  Serializer : MATLABFcn  MATLABFcn=repelem(u,d2dCfg.link.sps)
  Out1 : Outport
  wires:
  In1/1 -> FFEVector/1
  FFEVector/1 -> Serializer/1
  Serializer/1 -> DAC_Driver/1
  DAC_Driver/1 -> Out1/1, [txLane6_probe]

== system D2D_PHY_SI_Simulink/TX PMA x8/TX Lane 7 ==
  In1 : Inport
  DAC_Driver : MATLABFcn  MATLABFcn=dspPaperDriver(u,d2dCfg.txPma.lane)
  FFEVector : MATLABFcn  MATLABFcn=dspFfeVector(u,d2dCfg.txPma.lane.ffeCoeffs,d2dCfg.txPma.lane.ffeOffsets,struct('normalize',d2dCfg.txPma.lane.ffeNormalize,'currentConstraint',d2dCfg.txPma.lane.ffeCurrentConstraint))
  Serializer : MATLABFcn  MATLABFcn=repelem(u,d2dCfg.link.sps)
  Out1 : Outport
  wires:
  In1/1 -> FFEVector/1
  FFEVector/1 -> Serializer/1
  Serializer/1 -> DAC_Driver/1
  DAC_Driver/1 -> Out1/1, [txLane7_probe]

== system D2D_PHY_SI_Simulink/TX PMA x8/TX Lane 8 ==
  In1 : Inport
  DAC_Driver : MATLABFcn  MATLABFcn=dspPaperDriver(u,d2dCfg.txPma.lane)
  FFEVector : MATLABFcn  MATLABFcn=dspFfeVector(u,d2dCfg.txPma.lane.ffeCoeffs,d2dCfg.txPma.lane.ffeOffsets,struct('normalize',d2dCfg.txPma.lane.ffeNormalize,'currentConstraint',d2dCfg.txPma.lane.ffeCurrentConstraint))
  Serializer : MATLABFcn  MATLABFcn=repelem(u,d2dCfg.link.sps)
  Out1 : Outport
  wires:
  In1/1 -> FFEVector/1
  FFEVector/1 -> Serializer/1
  Serializer/1 -> DAC_Driver/1
  DAC_Driver/1 -> Out1/1, [txLane8_probe]
